simulink library "hrg_wa_v10_2_modules"  (R2025a)
settings: Solver=VariableStepAuto  StartTime=0.0  StopTime=10.0  RelTol=1e-3
undefined symbols (not defined in the file): Ad, Bd, p, x0
settings Model: Creator=11725  LastModifiedBy=11725

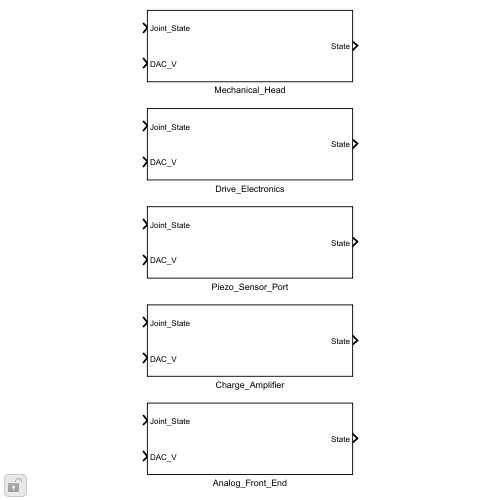
[thumbnail: Simulink's stored preview of the top-level diagram]
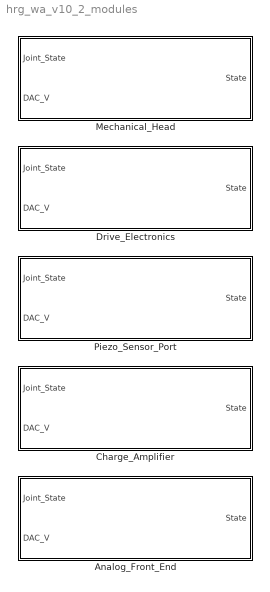
== system hrg_wa_v10_2_modules ==
  Analog_Front_End : Subsystem
  Charge_Amplifier : Subsystem
  Drive_Electronics : Subsystem
  Mechanical_Head : Subsystem
  Piezo_Sensor_Port : Subsystem

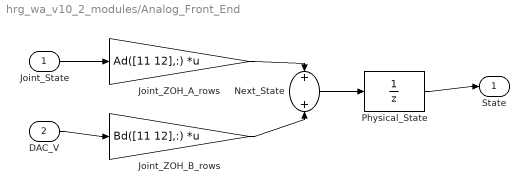
== system hrg_wa_v10_2_modules/Analog_Front_End ==
  Joint_State : Inport
  DAC_V : Inport  Port=2
  Joint_ZOH_A_rows : Gain  Gain=Ad([11 12],:)  Multiplication=Matrix(K*u)
  Joint_ZOH_B_rows : Gain  Gain=Bd([11 12],:)  Multiplication=Matrix(K*u)
  Next_State : Sum
  Physical_State : UnitDelay  InitialCondition=x0([11 12])  SampleTime=p.Ts  HasFrameUpgradeWarning=on
  State : Outport
  wires:
  Joint_State/1 -> Joint_ZOH_A_rows/1
  DAC_V/1 -> Joint_ZOH_B_rows/1
  Joint_ZOH_A_rows/1 -> Next_State/1
  Joint_ZOH_B_rows/1 -> Next_State/2
  Next_State/1 -> Physical_State/1
  Physical_State/1 -> State/1

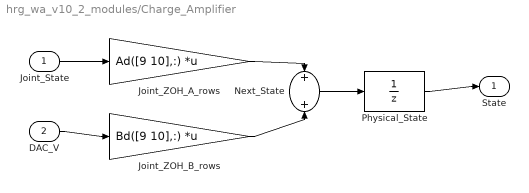
== system hrg_wa_v10_2_modules/Charge_Amplifier ==
  Joint_State : Inport
  DAC_V : Inport  Port=2
  Joint_ZOH_A_rows : Gain  Gain=Ad([9 10],:)  Multiplication=Matrix(K*u)
  Joint_ZOH_B_rows : Gain  Gain=Bd([9 10],:)  Multiplication=Matrix(K*u)
  Next_State : Sum
  Physical_State : UnitDelay  InitialCondition=x0([9 10])  SampleTime=p.Ts  HasFrameUpgradeWarning=on
  State : Outport
  wires:
  Joint_State/1 -> Joint_ZOH_A_rows/1
  DAC_V/1 -> Joint_ZOH_B_rows/1
  Joint_ZOH_A_rows/1 -> Next_State/1
  Joint_ZOH_B_rows/1 -> Next_State/2
  Next_State/1 -> Physical_State/1
  Physical_State/1 -> State/1

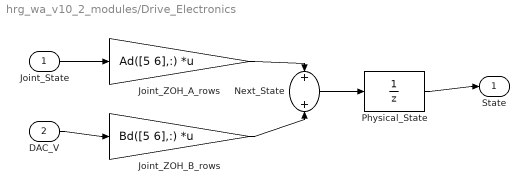
== system hrg_wa_v10_2_modules/Drive_Electronics ==
  Joint_State : Inport
  DAC_V : Inport  Port=2
  Joint_ZOH_A_rows : Gain  Gain=Ad([5 6],:)  Multiplication=Matrix(K*u)
  Joint_ZOH_B_rows : Gain  Gain=Bd([5 6],:)  Multiplication=Matrix(K*u)
  Next_State : Sum
  Physical_State : UnitDelay  InitialCondition=x0([5 6])  SampleTime=p.Ts  HasFrameUpgradeWarning=on
  State : Outport
  wires:
  Joint_State/1 -> Joint_ZOH_A_rows/1
  DAC_V/1 -> Joint_ZOH_B_rows/1
  Joint_ZOH_A_rows/1 -> Next_State/1
  Joint_ZOH_B_rows/1 -> Next_State/2
  Next_State/1 -> Physical_State/1
  Physical_State/1 -> State/1

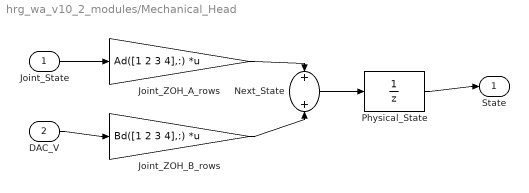
== system hrg_wa_v10_2_modules/Mechanical_Head ==
  Joint_State : Inport
  DAC_V : Inport  Port=2
  Joint_ZOH_A_rows : Gain  Gain=Ad([1 2 3 4],:)  Multiplication=Matrix(K*u)
  Joint_ZOH_B_rows : Gain  Gain=Bd([1 2 3 4],:)  Multiplication=Matrix(K*u)
  Next_State : Sum
  Physical_State : UnitDelay  InitialCondition=x0([1 2 3 4])  SampleTime=p.Ts  HasFrameUpgradeWarning=on
  State : Outport
  wires:
  Joint_State/1 -> Joint_ZOH_A_rows/1
  DAC_V/1 -> Joint_ZOH_B_rows/1
  Joint_ZOH_A_rows/1 -> Next_State/1
  Joint_ZOH_B_rows/1 -> Next_State/2
  Next_State/1 -> Physical_State/1
  Physical_State/1 -> State/1

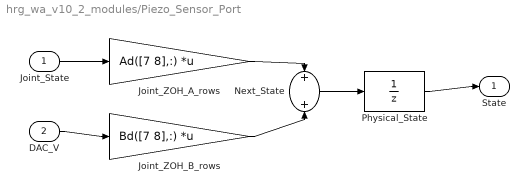
== system hrg_wa_v10_2_modules/Piezo_Sensor_Port ==
  Joint_State : Inport
  DAC_V : Inport  Port=2
  Joint_ZOH_A_rows : Gain  Gain=Ad([7 8],:)  Multiplication=Matrix(K*u)
  Joint_ZOH_B_rows : Gain  Gain=Bd([7 8],:)  Multiplication=Matrix(K*u)
  Next_State : Sum
  Physical_State : UnitDelay  InitialCondition=x0([7 8])  SampleTime=p.Ts  HasFrameUpgradeWarning=on
  State : Outport
  wires:
  Joint_State/1 -> Joint_ZOH_A_rows/1
  DAC_V/1 -> Joint_ZOH_B_rows/1
  Joint_ZOH_A_rows/1 -> Next_State/1
  Joint_ZOH_B_rows/1 -> Next_State/2
  Next_State/1 -> Physical_State/1
  Physical_State/1 -> State/1
